simulink model "Guidance_HIL_XPlane"  (R2026b)
settings: Solver=ode4  StopTime=80  FixedStep=0.005  MaxStep=0.05  MinStep=1e-8  AbsTol=1e-4
StartFcn:
  | ins_initial_state_xplane;
undefined symbols (not defined in the file or in its folder): sensors
(part 1 of 2)
settings Model: Creator=anade  LastModifiedBy=julio
settings DataIOCC: SaveState=on

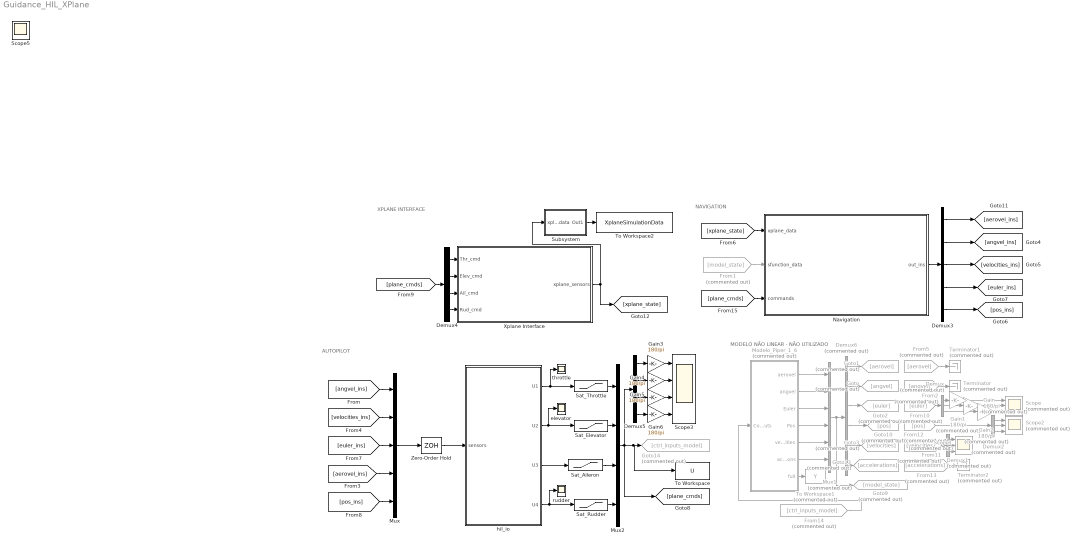
== system Guidance_HIL_XPlane ==
  note: MODELO NÃO LINEAR - NÃO UTILIZADO
  note: NAVIGATION
  note: AUTOPILOT
  note: XPLANE INTERFACE
  Demux : Demux  Commented=on  Outputs=3
  Demux1 : Demux  Commented=on  Outputs=3
  Demux2 : Demux  Commented=on  Outputs=3
  Demux3 : Demux  Outputs=5
  Demux4 : Demux
  Demux5 : Demux
  Demux6 : Demux  Commented=on  Outputs=6
  From1 : From  Commented=on  GotoTag=model_state
  From10 : From  Commented=on  GotoTag=euler
  From11 : From  Commented=on  GotoTag=velocities
  From12 : From  Commented=on  GotoTag=pos
  From13 : From  Commented=on  GotoTag=accelerations
  From14 : From  Commented=on  GotoTag=ctrl_inputs_model
  From2 : From  Commented=on  GotoTag=angvel
  From5 : From  Commented=on  GotoTag=aerovel
  Gain : Gain  Commented=on  Gain=180/pi
  Gain1 : Gain  Commented=on  Gain=180/pi
  Gain2 : Gain  Commented=on  Gain=180/pi
  Gain{3..6} (4 alike) : Gain  Gain=180/pi
  Goto : Goto  Commented=on  GotoTag=angvel
  Goto1 : Goto  Commented=on  GotoTag=aerovel
  Goto10 : Goto  Commented=on  GotoTag=pos
  Goto13 : Goto  Commented=on  GotoTag=accelerations
  Goto14 : Goto  Commented=on  GotoTag=ctrl_inputs_model
  Goto2 : Goto  Commented=on  GotoTag=euler
  Goto3 : Goto  Commented=on  GotoTag=velocities
  Goto9 : Goto  Commented=on  GotoTag=model_state
  Modelo_Piper_1_6 : Subsystem  Commented=on
  Mux : Mux  Inputs=5
  Mux1 : Mux  Commented=on  Inputs=6
  Mux2 : Mux
  Navigation : Subsystem
  Sat_Aileron : Saturate  UpperLimit=0.4363  LowerLimit=-0.4363
  Sat_Elevator : Saturate  UpperLimit=0.4363  LowerLimit=-0.4363
  Sat_Rudder : Saturate  UpperLimit=0.4363  LowerLimit=-0.4363
  Sat_Throttle : Saturate  UpperLimit=1  LowerLimit=0
  Scope : Scope  Commented=on  NumInputPorts=3
      settings: ActiveDisplayYMinimum=-6.98611  ActiveDisplayYMaximum=5.63762
  Scope1 : Scope  Commented=on  NumInputPorts=3
      settings: ActiveDisplayYMinimum=14.85385  ActiveDisplayYMaximum=15.01624
  Scope2 : Scope  Commented=on  NumInputPorts=3
      settings: ActiveDisplayYMinimum=-260.5736  ActiveDisplayYMaximum=2345.16236  DataLoggingVariableName=ScopeData4
  Scope3 : Scope  NumInputPorts=4
      settings: ActiveDisplayYMinimum=27.28743  ActiveDisplayYMaximum=28.20495
  Subsystem : Subsystem
  Terminator : Terminator  Commented=on
  Terminator1 : Terminator  Commented=on
  Terminator2 : Terminator  Commented=on
  To Workspace : ToWorkspace  VariableName=U  SaveFormat=Structure With Time  SampleTime=-1
  To Workspace1 : ToWorkspace  Commented=on  VariableName=Y  SaveFormat=Structure With Time  SampleTime=-1
  To Workspace2 : ToWorkspace  VariableName=XplaneSimulationData  SaveFormat=Structure With Time  SampleTime=-1
  Xplane Interface : Subsystem
  Zero-Order Hold : ZeroOrderHold  SampleTime=0.01
  elevator : Scope
      settings: ActiveDisplayYMinimum=-0.5444964451073081  ActiveDisplayYMaximum=0.59983808374051317  DataLoggingVariableName=ScopeData11
  hil_io : MATLAB Function  TreatAsAtomicUnit=on
  rudder : Scope
      settings: ActiveDisplayYMinimum=-0.082744402354985674  ActiveDisplayYMaximum=0.075589414066673855  DataLoggingVariableName=ScopeData9
  throttle : Scope
      settings: ActiveDisplayYMinimum=-0.079216538751602131  ActiveDisplayYMaximum=0.72681884876441949  DataLoggingVariableName=ScopeData10
  Scope5 : Scope
      settings: ActiveDisplayYMinimum=-10.063291139240507  ActiveDisplayYMaximum=10.936708860759492  DataLoggingVariableName=ScopeData6
  wires:
  Mux2/1 -> To Workspace/1, Goto14/1, [plane_cmds], Demux5/1
  Modelo_Piper_1_6/7(full) -> To Workspace1/1
  Demux/1 -> Gain1/1
  Demux/2 -> Gain/1
  Demux/3 -> Gain2/1
  Gain/1 -> Scope/2
  Demux1/1 -> Scope1/1
  Demux1/2 -> Scope1/2
  Demux1/3 -> Scope1/3
  Demux2/3 -> Scope2/3
  Demux2/2 -> Scope2/2
  Demux2/1 -> Scope2/1
  [aerovel_ins] -> Mux/4
  hil_io/1(U1) -> Sat_Throttle/1, throttle/1
  hil_io/2(U2) -> Sat_Elevator/1, elevator/1
  hil_io/3(U3) -> Sat_Aileron/1
  Gain1/1 -> Scope/1
  Gain2/1 -> Scope/3
  Gain3/1 -> Scope3/1
  Gain4/1 -> Scope3/2
  Gain5/1 -> Scope3/3
  Gain6/1 -> Scope3/4
  Sat_Throttle/1 -> Mux2/1
  Sat_Elevator/1 -> Mux2/2
  Sat_Aileron/1 -> Mux2/3
  Sat_Rudder/1 -> Mux2/4
  Demux3/2 -> [angvel_ins]
  Demux3/3 -> [velocities_ins]
  Demux3/4 -> [euler_ins]
  Demux3/5 -> [pos_ins]
  Navigation/1(out_ins) -> Demux3/1
  [angvel_ins] -> Mux/1
  [velocities_ins] -> Mux/2
  [euler_ins] -> Mux/3
  [pos_ins] -> Mux/5
  [plane_cmds] -> Demux4/1
  Demux4/1 -> Xplane Interface/1(Thr_cmd)
  Demux4/2 -> Xplane Interface/2(Elev_cmd)
  Demux4/3 -> Xplane Interface/3(Ail_cmd)
  Demux4/4 -> Xplane Interface/4(Rud_cmd)
  Demux5/1 -> Gain3/1
  Demux5/2 -> Gain4/1
  Demux5/3 -> Gain5/1
  Demux5/4 -> Gain6/1
  Modelo_Piper_1_6/1(aerovel) -> Mux1/1
  Modelo_Piper_1_6/2(angvel) -> Mux1/2
  Modelo_Piper_1_6/3(Euler) -> Mux1/3
  Modelo_Piper_1_6/4(Pos) -> Mux1/4
  Modelo_Piper_1_6/5(velocities) -> Mux1/5
  Demux6/1 -> Goto1/1
  Demux6/2 -> Goto/1
  Demux6/3 -> Goto2/1
  Demux6/4 -> Goto10/1
  Demux6/5 -> Goto3/1
  From2/1 -> Terminator/1
  Demux3/1 -> [aerovel_ins]
  From5/1 -> Terminator1/1
  From12/1 -> Demux2/1
  From10/1 -> Demux/1
  From11/1 -> Demux1/1
  Xplane Interface/1(xplane_sensors) -> Subsystem/1(xplane_data), [xplane_state]
  [xplane_state] -> Navigation/1(xplane_data)
  Modelo_Piper_1_6/6(accelerations) -> Mux1/6
  Mux1/1 -> Goto9/1, Demux6/1
  Demux6/6 -> Goto13/1
  From13/1 -> Terminator2/1
  hil_io/4(U4) -> Sat_Rudder/1, rudder/1
  Subsystem/1(Out1) -> To Workspace2/1
  From14/1 -> Modelo_Piper_1_6/1(Control Inputs)
  From1/1 -> Navigation/2(sfunction_data)
  [plane_cmds] -> Navigation/3(commands)
  Zero-Order Hold/1 -> hil_io/1(sensors)
  Mux/1 -> Zero-Order Hold/1

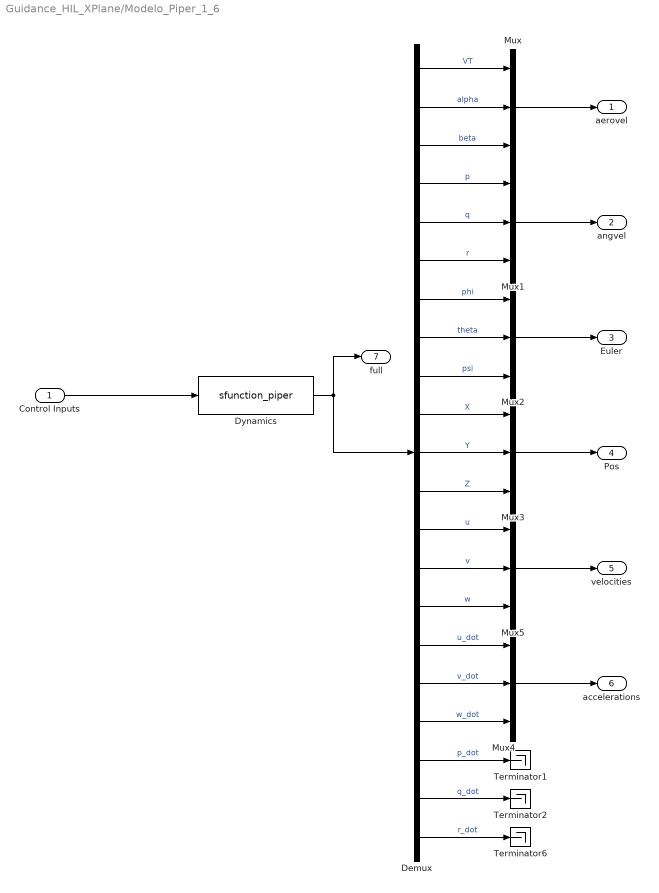
== system Guidance_HIL_XPlane/Modelo_Piper_1_6 ==
  Control Inputs : Inport
  Demux : Demux  Outputs=21
  Dynamics : S-Function  FunctionName=sfunction_piper  Parameters=par_gen,par_aero,par_prop, Xe  SFunctionDeploymentMode=off  EnableBusSupport=off
  Mux{,1..5} (6 alike) : Mux  Inputs=3
  Terminator1 : Terminator
  Terminator2 : Terminator
  Terminator6 : Terminator
  aerovel : Outport
  angvel : Outport  Port=2
  Euler : Outport  Port=3
  Pos : Outport  Port=4
  velocities : Outport  Port=5
  accelerations : Outport  Port=6
  full : Outport  Port=7
  wires:
  Control Inputs/1 -> Dynamics/1
  Dynamics/1 -> full/1, Demux/1
  Demux/1 -> Mux/1  "VT"
  Demux/2 -> Mux/2  "alpha"
  Demux/3 -> Mux/3  "beta"
  Mux/1 -> aerovel/1
  Demux/6 -> Mux1/3  "r"
  Demux/4 -> Mux1/1  "p"
  Mux1/1 -> angvel/1
  Demux/5 -> Mux1/2  "q"
  Mux2/1 -> Euler/1
  Demux/9 -> Mux2/3  "psi"
  Demux/7 -> Mux2/1  "phi"
  Demux/8 -> Mux2/2  "theta"
  Demux/11 -> Mux3/2  "Y"
  Demux/10 -> Mux3/1  "X"
  Demux/12 -> Mux3/3  "Z"
  Mux3/1 -> Pos/1
  Demux/14 -> Mux5/2  "v"
  Demux/15 -> Mux5/3  "w"
  Demux/17 -> Mux4/2  "v_dot"
  Demux/18 -> Mux4/3  "w_dot"
  Demux/16 -> Mux4/1  "u_dot"
  Demux/19 -> Terminator1/1  "p_dot"
  Demux/20 -> Terminator2/1  "q_dot"
  Demux/21 -> Terminator6/1  "r_dot"
  Demux/13 -> Mux5/1  "u"
  Mux5/1 -> velocities/1
  Mux4/1 -> accelerations/1

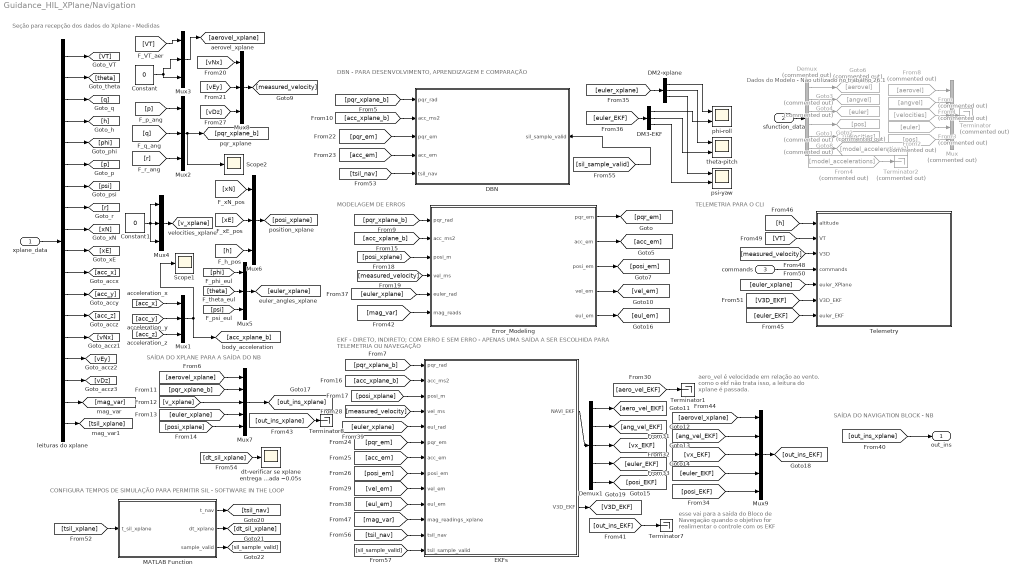
== system Guidance_HIL_XPlane/Navigation ==
  note: CONFIGURA TEMPOS DE SIMULAÇÃO PARA PERMITIR
      | SIL - SOFTWARE IN THE LOOP
  note: DBN - PARA DESENVOLVIMENTO, APRENDIZAGEM E COMPARAÇÃO
  note: MODELAGEM DE ERROS
  note: EKF - DIRETO, INDIRETO; COM ERRO E SEM ERRO - APENAS UMA SAÍDA A SER ESCOLHIDA PARA TELEMETRIA OU NAVEGAÇÃO
  note: TELEMETRIA PARA O CLI
  note: aero_vel é velocidade em relação ao vento.
      | como o ekf não trata isso, a leitura do xplane é passada.
  note: SAÍDA DO NAVIGATION BLOCK - NB
  note: SAÍDA DO XPLANE PARA A SAÍDA DO NB
  note: Seção para recepção dos dados do Xplane - Medidas
  note: Dados do Modelo - Não utilizado no trabalho 26.1
  note: esse vai para a saída do
      | Bloco de Navegação quando o objetivo
      | for realimentar o controle com os EKF
  xplane_data : Inport
  sfunction_data : Inport  Port=2
  commands : Inport  Port=3
  Constant : Constant  Value=0
  Constant1 : Constant  Value=0
  DBN : Subsystem
      settings: PortSchema="{\"entries\":[{\"content\":{\"sides\":[{\"content\":{\"connectorIds\":[\"In1\",\"In2\",\"In3\",\"In4\",\"In5\"]},\"type\":\"ConnectorPlacement.EquallySpacedRectSide\",\"uuid\":\"e1d6fc02-7142-43fa-9a22-3751041ad3ea\"},{\"content\":{\"connectorIds\":[\"In6\"],\"side\":\"RIGHT\"},\"type\":\"ConnectorPlacement.EquallySpacedRectSide\",\"uuid\":\"c1701565-012f-4813-aa31-4d1b787e29e9\"},{\"content\":{\"side\":\"TOP\"},\"type\":\"ConnectorPlacement.EquallySpacedRectSide\",\"uuid\":\"7000accd-9525-4039-8d3a-2953233d8ced\"},{\"content\":{\"side\":\"BOTTOM\"},\"type\":\"ConnectorPlacement.EquallySpacedRectSide\",\"uuid\":\"71202a87-1554-4160-a726-314bf509973f\"}]},\"type\":\"ConnectorPlacement.EquallySpacedConnector\",\"uuid\":\"ce59d3ba-4702-4e8e-9706-d7679f847eab\"}],\"packageUris\":[\"http://schema.mathworks.com/mf0/Connector/R2020b\"],\"version\":\"1.0\"}"
  DM2-xplane : Demux  Outputs=3
  DM3-EKF : Demux  Outputs=3
  Demux : Demux  Commented=on  Outputs=6
  Demux1 : Demux  Outputs=5
  EKFs : Subsystem
  Error_Modeling : Subsystem
  From : From  Commented=on  GotoTag=angvel
  From1 : From  Commented=on  GotoTag=velocities
  From2 : From  Commented=on  GotoTag=euler
  From3 : From  Commented=on  GotoTag=pos
  From4 : From  Commented=on  GotoTag=model_accelerations
  From8 : From  Commented=on  GotoTag=aerovel
  Goto1 : Goto  Commented=on  GotoTag=velocities
  Goto2 : Goto  Commented=on  GotoTag=pos
  Goto3 : Goto  Commented=on  GotoTag=angvel
  Goto4 : Goto  Commented=on  GotoTag=euler
  Goto6 : Goto  Commented=on  GotoTag=aerovel
  Goto8 : Goto  Commented=on  GotoTag=model_accelerations
  MATLAB Function : MATLAB Function  TreatAsAtomicUnit=on
  Mux : Mux  Commented=on  Inputs=5
  Mux{1..6,8} (7 alike) : Mux  Inputs=3
  Mux7 : Mux  Inputs=5
  Mux9 : Mux  Inputs=5
  Scope1 : Scope
      settings: ActiveDisplayYMinimum=-16.174539597742694  ActiveDisplayYMaximum=12.212616009640644  DataLoggingVariableName=ScopeData7
  Scope2 : Scope
      settings: DataLoggingVariableName=ScopeData8
  Telemetry : Subsystem
  Terminator : Terminator  Commented=on
  Terminator1 : Terminator
  Terminator2 : Terminator  Commented=on
  Terminator7 : Terminator
  Terminator8 : Terminator
  dt-verificar se xplane entrega a cada ~0.05s : Scope
      settings: ActiveDisplayYMinimum=-39.174751163951377  ActiveDisplayYMaximum=35.494375282880192  DataLoggingVariableName=ScopeData18
  leituras do xplane : Demux  Outputs=18
  phi-roll : Scope  NumInputPorts=2
      settings: ActiveDisplayYMinimum=-36.313013678398512  ActiveDisplayYMaximum=32.517817448050167  DataLoggingVariableName=ScopeData13
  psi-yaw : Scope  NumInputPorts=2
      settings: ActiveDisplayYMinimum=-3.9264088034500482  ActiveDisplayYMaximum=3.9263427428668405  DataLoggingVariableName=ScopeData17
  theta-pitch : Scope  NumInputPorts=2
      settings: ActiveDisplayYMinimum=-1.9059189366815974  ActiveDisplayYMaximum=3.346694670659121  DataLoggingVariableName=ScopeData16
  out_ins : Outport
  wires:
  xplane_data/1 -> leituras do xplane/1
  leituras do xplane/1 -> [VT]
  leituras do xplane/6 -> [p]
  leituras do xplane/9 -> [xN]
  leituras do xplane/3 -> [q]
  leituras do xplane/8 -> [r]
  leituras do xplane/5 -> [phi]
  leituras do xplane/10 -> [xE]
  leituras do xplane/2 -> [theta]
  leituras do xplane/7 -> [psi]
  leituras do xplane/4 -> [h]
  leituras do xplane/11 -> [acc_x]
  leituras do xplane/12 -> [acc_y]
  leituras do xplane/13 -> [acc_z]
  [VT] -> Mux3/1
  [p] -> Mux2/1
  [r] -> Mux2/3
  [acc_x] -> Mux1/1
  [acc_y] -> Mux1/2
  [acc_z] -> Mux1/3
  Mux1/1 -> Scope1/1, [acc_xplane_b]
  Mux2/1 -> [pqr_xplane_b], Scope2/1
  [q] -> Mux2/2
  Constant/1 -> Mux3/2, Mux3/3
  Mux3/1 -> [aerovel_xplane]
  Constant1/1 -> Mux4/3, Mux4/1, Mux4/2
  Mux4/1 -> [v_xplane]
  Mux5/1 -> [euler_xplane]
  [phi] -> Mux5/1
  [theta] -> Mux5/2
  [psi] -> Mux5/3
  [xN] -> Mux6/1
  [xE] -> Mux6/2
  [h] -> Mux6/3
  Mux6/1 -> [posi_xplane]
  [aerovel_xplane] -> Mux7/1
  [pqr_xplane_b] -> Mux7/2
  [v_xplane] -> Mux7/3
  [euler_xplane] -> Mux7/4
  [posi_xplane] -> Mux7/5
  [pqr_xplane_b] -> DBN/1(pqr_rad)
  [acc_xplane_b] -> DBN/2(acc_ms2)
  Error_Modeling/1(pqr_em) -> [pqr_em]
  Error_Modeling/2(acc_em) -> [acc_em]
  Error_Modeling/3(posi_em) -> [posi_em]
  [pqr_xplane_b] -> EKFs/1(pqr_rad)
  [acc_xplane_b] -> EKFs/2(acc_ms2)
  [posi_xplane] -> EKFs/3(posi_m)
  [pqr_xplane_b] -> Error_Modeling/1(pqr_rad)
  [acc_xplane_b] -> Error_Modeling/2(acc_ms2)
  [posi_xplane] -> Error_Modeling/3(posi_m)
  [pqr_em] -> DBN/3(pqr_em)
  [acc_em] -> DBN/4(acc_em)
  [measured_velocity] -> EKFs/4(vel_ms)
  [pqr_em] -> EKFs/6(pqr_em)
  [acc_em] -> EKFs/7(acc_em)
  [posi_em] -> EKFs/8(posi_em)
  leituras do xplane/14 -> [vNx]
  leituras do xplane/15 -> [vEy]
  leituras do xplane/16 -> [vDz]
  [vNx] -> Mux8/1
  [vEy] -> Mux8/2
  [vDz] -> Mux8/3
  Mux8/1 -> [measured_velocity]
  [measured_velocity] -> Error_Modeling/4(vel_ms)
  Error_Modeling/4(vel_em) -> [vel_em]
  [vel_em] -> EKFs/9(vel_em)
  Demux1/1 -> [aero_vel_EKF]
  Demux1/2 -> [ang_vel_EKF]
  Demux1/3 -> [vx_EKF]
  Demux1/4 -> [euler_EKF]
  Demux1/5 -> [posi_EKF]
  [aero_vel_EKF] -> Terminator1/1
  [ang_vel_EKF] -> Mux9/2
  [vx_EKF] -> Mux9/3
  [euler_EKF] -> Mux9/4
  [posi_EKF] -> Mux9/5
  [euler_xplane] -> DM2-xplane/1
  DM2-xplane/1 -> phi-roll/1
  DM2-xplane/2 -> theta-pitch/1
  DM2-xplane/3 -> psi-yaw/1
  [euler_EKF] -> DM3-EKF/1
  DM3-EKF/1 -> phi-roll/2
  DM3-EKF/2 -> theta-pitch/2
  DM3-EKF/3 -> psi-yaw/2
  Demux/5 -> Goto1/1
  Mux/1 -> Terminator/1
  From8/1 -> Mux/1
  Demux/6 -> Goto8/1
  Demux/1 -> Goto6/1
  Demux/2 -> Goto3/1
  From/1 -> Mux/2
  From3/1 -> Mux/5
  From4/1 -> Terminator2/1
  Demux/3 -> Goto4/1
  From2/1 -> Mux/4
  Demux/4 -> Goto2/1
  From1/1 -> Mux/3
  sfunction_data/1 -> Demux/1
  [euler_xplane] -> Error_Modeling/5(euler_rad)
  Error_Modeling/5(eul_em) -> [eul_em]
  [eul_em] -> EKFs/10(eul_em)
  [euler_xplane] -> EKFs/5(eul_rad)
  Mux7/1 -> [out_ins_xplane]
  [out_ins_xplane] -> out_ins/1
  EKFs/1(NAVI_EKF) -> Demux1/1
  [out_ins_EKF] -> Terminator7/1
  [out_ins_xplane] -> Terminator8/1
  leituras do xplane/17 -> [mag_var]
  [mag_var] -> EKFs/11(mag_readings_xplane)
  [mag_var] -> Error_Modeling/6(mag_reads)
  Mux9/1 -> [out_ins_EKF]
  [aerovel_xplane] -> Mux9/1
  commands/1 -> Telemetry/4(commands)
  [h] -> Telemetry/1(altitude)
  [measured_velocity] -> Telemetry/3(V3D)
  [VT] -> Telemetry/2(VT)
  [euler_xplane] -> Telemetry/5(euler_XPlane)
  [euler_EKF] -> Telemetry/7(euler_EKF)
  EKFs/2(V3D_EKF) -> [V3D_EKF]
  [V3D_EKF] -> Telemetry/6(V3D_EKF)
  leituras do xplane/18 -> [tsil_xplane]
  [tsil_xplane] -> MATLAB Function/1(t_sil_xplane)
  MATLAB Function/2(dt_xplane) -> [dt_sil_xplane]
  MATLAB Function/1(t_nav) -> [tsil_nav]
  MATLAB Function/3(sample_valid) -> [sil_sample_valid]
  [tsil_nav] -> DBN/5(tsil_nav)
  [sil_sample_valid] -> DBN/6(sil_sample_valid)
  [dt_sil_xplane] -> dt-verificar se xplane entrega a cada ~0.05s/1
  [tsil_nav] -> EKFs/12(tsil_nav)
  [sil_sample_valid] -> EKFs/13(tsil_sample_valid)

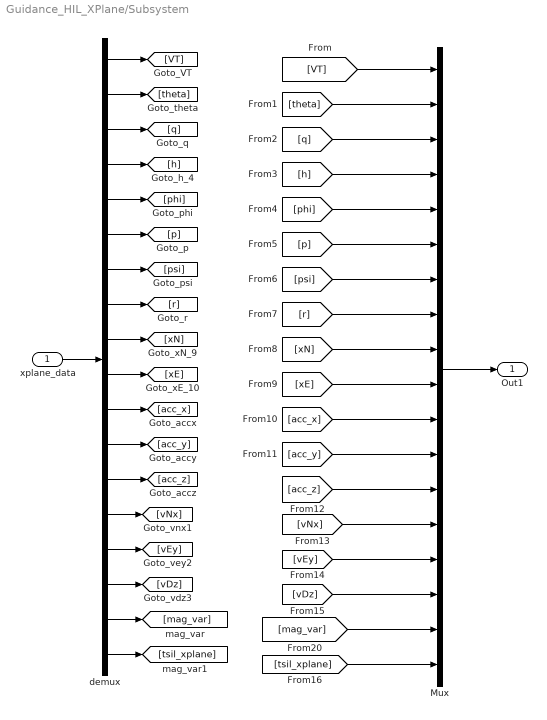
== system Guidance_HIL_XPlane/Subsystem ==
  xplane_data : Inport
  Mux : Mux  Inputs=18
  demux : Demux  Outputs=18
  Out1 : Outport
  wires:
  demux/3 -> [q]
  demux/8 -> [r]
  demux/4 -> [h]
  demux/2 -> [theta]
  demux/6 -> [p]
  demux/1 -> [VT]
  xplane_data/1 -> demux/1
  demux/9 -> [xN]
  demux/12 -> [acc_y]
  demux/11 -> [acc_x]
  demux/13 -> [acc_z]
  demux/10 -> [xE]
  demux/7 -> [psi]
  demux/5 -> [phi]
  [VT] -> Mux/1
  [theta] -> Mux/2
  [q] -> Mux/3
  [h] -> Mux/4
  [phi] -> Mux/5
  [p] -> Mux/6
  [psi] -> Mux/7
  [r] -> Mux/8
  [xN] -> Mux/9
  [xE] -> Mux/10
  [acc_x] -> Mux/11
  [acc_y] -> Mux/12
  [acc_z] -> Mux/13
  Mux/1 -> Out1/1
  demux/14 -> [vNx]
  demux/15 -> [vEy]
  demux/16 -> [vDz]
  [vNx] -> Mux/14
  [vEy] -> Mux/15
  [vDz] -> Mux/16
  [mag_var] -> Mux/17
  demux/17 -> [mag_var]
  demux/18 -> [tsil_xplane]
  [tsil_xplane] -> Mux/18

== system Guidance_HIL_XPlane/Xplane Interface ==
  Thr_cmd : Inport
  Elev_cmd : Inport  Port=2
  Ail_cmd : Inport  Port=3
  Rud_cmd : Inport  Port=4
  Clock : Clock
  Cmd Mux : Mux
  Terminator : Terminator
  X-Plane Actuators : MATLAB Function  TreatAsAtomicUnit=on
  X-Plane Sensors : MATLAB Function  TreatAsAtomicUnit=on
  Zero-Order Hold : ZeroOrderHold  SampleTime=0.01
  xplane_sensors : Outport
  wires:
  Cmd Mux/1 -> Zero-Order Hold/1
  Elev_cmd/1 -> Cmd Mux/1
  Ail_cmd/1 -> Cmd Mux/2
  Rud_cmd/1 -> Cmd Mux/3
  Thr_cmd/1 -> Cmd Mux/4
  Clock/1 -> X-Plane Sensors/1(t), X-Plane Actuators/2(t)
  X-Plane Actuators/1(status) -> Terminator/1
  Zero-Order Hold/1 -> X-Plane Actuators/1(u)
  X-Plane Sensors/1(xplane_sensors) -> xplane_sensors/1

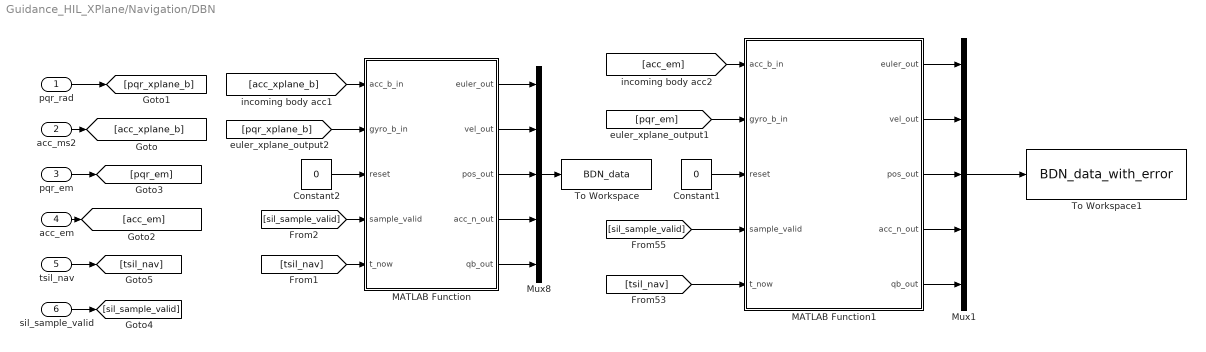
== system Guidance_HIL_XPlane/Navigation/DBN ==
  pqr_rad : Inport
  acc_ms2 : Inport  Port=2
  pqr_em : Inport  Port=3
  acc_em : Inport  Port=4
  tsil_nav : Inport  Port=5
  sil_sample_valid : Inport  Port=6
  Constant1 : Constant  Value=0
  Constant2 : Constant  Value=0
  MATLAB Function : MATLAB Function  TreatAsAtomicUnit=on
  MATLAB Function1 : MATLAB Function  TreatAsAtomicUnit=on
  Mux1 : Mux  Inputs=5
  Mux8 : Mux  Inputs=5
  To Workspace : ToWorkspace  VariableName=BDN_data  SaveFormat=Structure With Time  SampleTime=-1
  To Workspace1 : ToWorkspace  VariableName=BDN_data_with_error  SaveFormat=Structure With Time  SampleTime=-1
  wires:
  Constant2/1 -> MATLAB Function/3(reset)
  MATLAB Function/2(vel_out) -> Mux8/2
  MATLAB Function/1(euler_out) -> Mux8/1
  MATLAB Function/4(acc_n_out) -> Mux8/4
  MATLAB Function/5(qb_out) -> Mux8/5
  MATLAB Function/3(pos_out) -> Mux8/3
  Mux8/1 -> To Workspace/1
  [acc_xplane_b] -> MATLAB Function/1(acc_b_in)
  [pqr_xplane_b] -> MATLAB Function/2(gyro_b_in)
  acc_ms2/1 -> [acc_xplane_b]
  pqr_rad/1 -> [pqr_xplane_b]
  [pqr_em] -> MATLAB Function1/2(gyro_b_in)
  [acc_em] -> MATLAB Function1/1(acc_b_in)
  [tsil_nav] -> MATLAB Function1/5(t_now)
  Mux1/1 -> To Workspace1/1
  MATLAB Function1/3(pos_out) -> Mux1/3
  MATLAB Function1/5(qb_out) -> Mux1/5
  MATLAB Function1/2(vel_out) -> Mux1/2
  MATLAB Function1/4(acc_n_out) -> Mux1/4
  [sil_sample_valid] -> MATLAB Function1/4(sample_valid)
  MATLAB Function1/1(euler_out) -> Mux1/1
  Constant1/1 -> MATLAB Function1/3(reset)
  acc_em/1 -> [acc_em]
  pqr_em/1 -> [pqr_em]
  sil_sample_valid/1 -> [sil_sample_valid]
  tsil_nav/1 -> [tsil_nav]
  [tsil_nav] -> MATLAB Function/5(t_now)
  [sil_sample_valid] -> MATLAB Function/4(sample_valid)

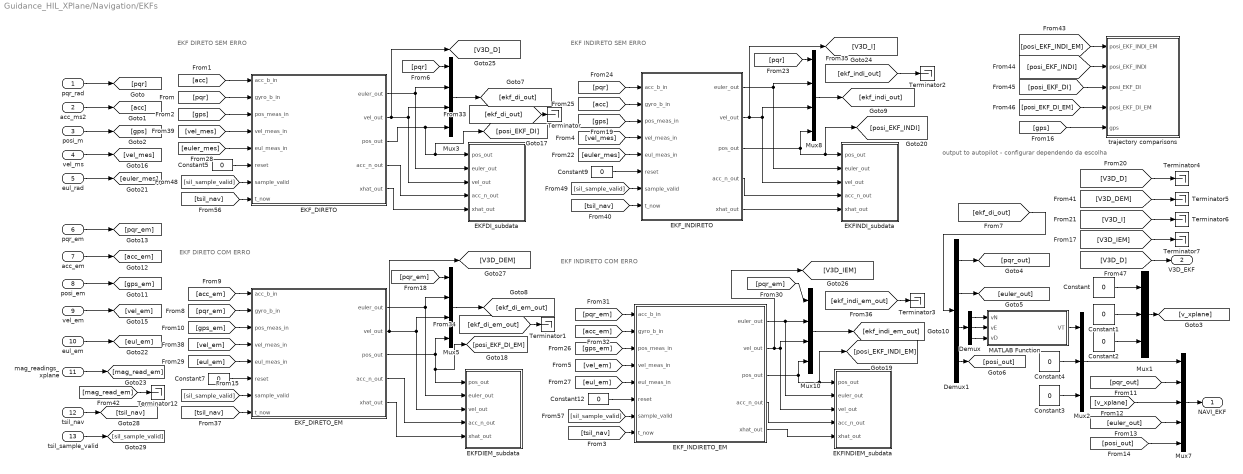
== system Guidance_HIL_XPlane/Navigation/EKFs ==
  note: EKF INDIRETO COM ERRO
  note: EKF INDIRETO SEM ERRO
  note: EKF DIRETO COM ERRO
  note: EKF DIRETO SEM ERRO
  note: output to autopilot - configurar dependendo da escolha
  pqr_rad : Inport
  acc_ms2 : Inport  Port=2
  posi_m : Inport  Port=3
  vel_ms : Inport  Port=4
  eul_rad : Inport  Port=5
  pqr_em : Inport  Port=6
  acc_em : Inport  Port=7
  posi_em : Inport  Port=8
  vel_em : Inport  Port=9
  eul_em : Inport  Port=10
  mag_readings_xplane : Inport  Port=11
  tsil_nav : Inport  Port=12
  tsil_sample_valid : Inport  Port=13
  Constant{,1..5,7,9,12} (9 alike) : Constant  Value=0
  Demux : Demux  Outputs=3
  Demux1 : Demux
  EKFDIEM_subdata : Subsystem
  EKFDI_subdata : Subsystem
  EKFINDIEM_subdata : Subsystem
  EKFINDI_subdata : Subsystem
  EKF_DIRETO : MATLAB Function  TreatAsAtomicUnit=on
  EKF_DIRETO_EM : MATLAB Function  TreatAsAtomicUnit=on
  EKF_INDIRETO : MATLAB Function  TreatAsAtomicUnit=on
  EKF_INDIRETO_EM : MATLAB Function  TreatAsAtomicUnit=on
  MATLAB Function : MATLAB Function  TreatAsAtomicUnit=on
  Mux1 : Mux  Inputs=3
  Mux{3,5,8,10} (4 alike) : Mux
  Mux2 : Mux  Inputs=3
  Mux7 : Mux  Inputs=5
  Terminator{,1..7,12} (9 alike) : Terminator
  trajectory comparisons : Subsystem
  NAVI_EKF : Outport
  V3D_EKF : Outport  Port=2
  wires:
  EKF_DIRETO/3(pos_out) -> Mux3/4, EKFDI_subdata/1(pos_out), [posi_EKF_DI]
  posi_m/1 -> [gps]
  acc_ms2/1 -> [acc]
  pqr_rad/1 -> [pqr]
  [gps] -> EKF_DIRETO/3(pos_meas_in)
  Mux7/1 -> NAVI_EKF/1
  [posi_out] -> Mux7/5
  [v_xplane] -> Mux7/3
  [pqr_out] -> Mux7/2
  [euler_out] -> Mux7/4
  Mux1/1 -> [v_xplane]
  Constant/1 -> Mux1/1
  Constant2/1 -> Mux1/3
  Constant1/1 -> Mux1/2
  Demux/1 -> MATLAB Function/1(vN)
  Demux/2 -> MATLAB Function/2(vE)
  Demux/3 -> MATLAB Function/3(vD)
  MATLAB Function/1(VT) -> Mux2/1
  Constant4/1 -> Mux2/2
  Constant3/1 -> Mux2/3
  Mux2/1 -> Mux7/1
  Demux1/4 -> [posi_out]
  Mux3/1 -> [ekf_di_out]
  [ekf_di_out] -> Demux1/1
  [gps_em] -> EKF_DIRETO_EM/3(pos_meas_in)
  EKF_DIRETO_EM/3(pos_out) -> [posi_EKF_DI_EM], EKFDIEM_subdata/1(pos_out), Mux5/4
  EKF_DIRETO_EM/1(euler_out) -> Mux5/2, EKFDIEM_subdata/2(euler_out)
  Mux5/1 -> [ekf_di_em_out]
  Mux8/1 -> [ekf_indi_out]
  [pqr] -> EKF_INDIRETO/1(acc_b_in)
  EKF_INDIRETO/3(pos_out) -> Mux8/4, [posi_EKF_INDI], EKFINDI_subdata/1(pos_out)
  [gps] -> EKF_INDIRETO/3(pos_meas_in)
  [acc] -> EKF_INDIRETO/2(gyro_b_in)
  [acc_em] -> EKF_INDIRETO_EM/2(gyro_b_in)
  [gps_em] -> EKF_INDIRETO_EM/3(pos_meas_in)
  [pqr_em] -> EKF_INDIRETO_EM/1(acc_b_in)
  Mux10/1 -> [ekf_indi_em_out]
  [ekf_di_out] -> Terminator/1
  [ekf_di_em_out] -> Terminator1/1
  [ekf_indi_out] -> Terminator2/1
  [ekf_indi_em_out] -> Terminator3/1
  [tsil_nav] -> EKF_DIRETO/8(t_now)
  Constant5/1 -> EKF_DIRETO/6(reset)
  pqr_em/1 -> [pqr_em]
  acc_em/1 -> [acc_em]
  posi_em/1 -> [gps_em]
  vel_em/1 -> [vel_em]
  vel_ms/1 -> [vel_mes]
  [vel_mes] -> EKF_DIRETO/4(vel_meas_in)
  [acc_em] -> EKF_DIRETO_EM/1(acc_b_in)
  [pqr_em] -> EKF_DIRETO_EM/2(gyro_b_in)
  [vel_em] -> EKF_DIRETO_EM/4(vel_meas_in)
  [pqr] -> EKF_DIRETO/2(gyro_b_in)
  [acc] -> EKF_DIRETO/1(acc_b_in)
  Constant7/1 -> EKF_DIRETO_EM/6(reset)
  EKF_DIRETO/4(acc_n_out) -> EKFDI_subdata/4(acc_n_out)
  EKF_DIRETO/5(xhat_out) -> EKFDI_subdata/5(xhat_out)
  [pqr] -> Mux3/1
  EKF_DIRETO/1(euler_out) -> Mux3/2, EKFDI_subdata/2(euler_out)
  EKF_DIRETO/2(vel_out) -> [V3D_D], Mux3/3, EKFDI_subdata/3(vel_out)
  EKF_DIRETO_EM/5(xhat_out) -> EKFDIEM_subdata/5(xhat_out)
  Demux1/3 -> Demux/1
  Demux1/1 -> [pqr_out]
  Demux1/2 -> [euler_out]
  [pqr_em] -> Mux5/1
  EKF_DIRETO_EM/2(vel_out) -> Mux5/3, EKFDIEM_subdata/3(vel_out), [V3D_DEM]
  EKF_DIRETO_EM/4(acc_n_out) -> EKFDIEM_subdata/4(acc_n_out)
  [pqr] -> Mux8/1
  Constant9/1 -> EKF_INDIRETO/6(reset)
  [vel_mes] -> EKF_INDIRETO/4(vel_meas_in)
  EKF_INDIRETO/5(xhat_out) -> EKFINDI_subdata/5(xhat_out)
  EKF_INDIRETO/4(acc_n_out) -> EKFINDI_subdata/4(acc_n_out)
  EKF_INDIRETO/1(euler_out) -> Mux8/2, EKFINDI_subdata/2(euler_out)
  EKF_INDIRETO/2(vel_out) -> [V3D_I], Mux8/3, EKFINDI_subdata/3(vel_out)
  [pqr_em] -> Mux10/1
  EKF_INDIRETO_EM/1(euler_out) -> Mux10/2, EKFINDIEM_subdata/2(euler_out)
  EKF_INDIRETO_EM/2(vel_out) -> [V3D_IEM], Mux10/3, EKFINDIEM_subdata/3(vel_out)
  EKF_INDIRETO_EM/3(pos_out) -> Mux10/4, [posi_EKF_INDI_EM], EKFINDIEM_subdata/1(pos_out)
  [vel_em] -> EKF_INDIRETO_EM/4(vel_meas_in)
  Constant12/1 -> EKF_INDIRETO_EM/6(reset)
  EKF_INDIRETO_EM/4(acc_n_out) -> EKFINDIEM_subdata/4(acc_n_out)
  EKF_INDIRETO_EM/5(xhat_out) -> EKFINDIEM_subdata/5(xhat_out)
  eul_rad/1 -> [euler_mes]
  eul_em/1 -> [eul_em]
  [euler_mes] -> EKF_DIRETO/5(eul_meas_in)
  [eul_em] -> EKF_DIRETO_EM/5(eul_meas_in)
  [euler_mes] -> EKF_INDIRETO/5(eul_meas_in)
  [eul_em] -> EKF_INDIRETO_EM/5(eul_meas_in)
  mag_readings_xplane/1 -> [mag_read_em]
  [mag_read_em] -> Terminator12/1
  [posi_EKF_INDI_EM] -> trajectory comparisons/1(posi_EKF_INDI_EM)
  [posi_EKF_INDI] -> trajectory comparisons/2(posi_EKF_INDI)
  [posi_EKF_DI] -> trajectory comparisons/3(posi_EKF_DI)
  [posi_EKF_DI_EM] -> trajectory comparisons/4(posi_EKF_DI_EM)
  [gps] -> trajectory comparisons/5(gps)
  [V3D_D] -> Terminator4/1
  [V3D_DEM] -> Terminator5/1
  [V3D_I] -> Terminator6/1
  [V3D_IEM] -> Terminator7/1
  [V3D_D] -> V3D_EKF/1
  tsil_nav/1 -> [tsil_nav]
  tsil_sample_valid/1 -> [sil_sample_valid]
  [tsil_nav] -> EKF_DIRETO_EM/8(t_now)
  [tsil_nav] -> EKF_INDIRETO/8(t_now)
  [sil_sample_valid] -> EKF_INDIRETO_EM/7(sample_valid)
  [tsil_nav] -> EKF_INDIRETO_EM/8(t_now)
  [sil_sample_valid] -> EKF_DIRETO_EM/7(sample_valid)
  [sil_sample_valid] -> EKF_DIRETO/7(sample_valid)
  [sil_sample_valid] -> EKF_INDIRETO/7(sample_valid)

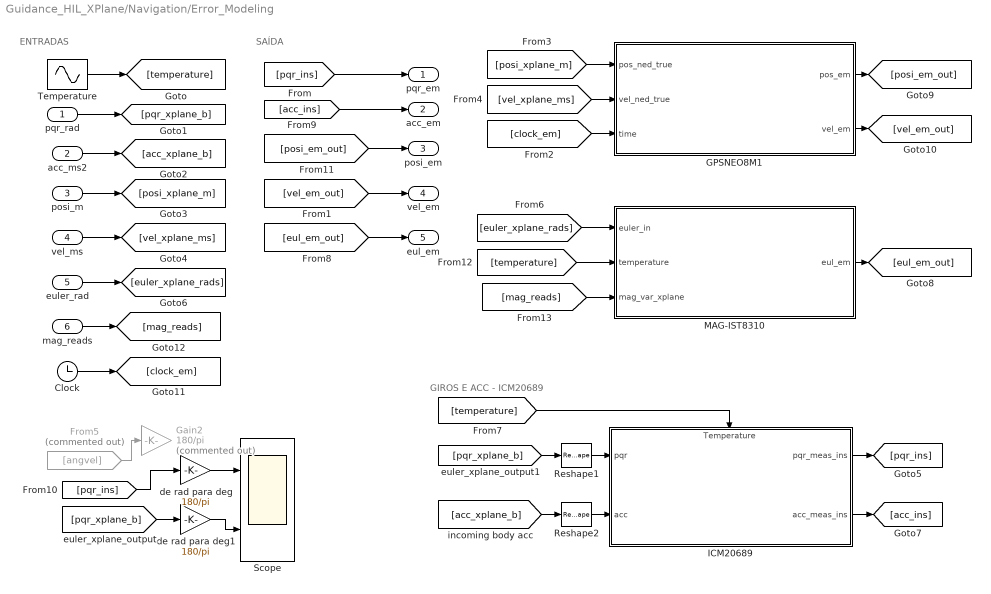
== system Guidance_HIL_XPlane/Navigation/Error_Modeling ==
  note: GIROS E ACC - ICM20689
  note: ENTRADAS
  note: SAÍDA
  pqr_rad : Inport
  acc_ms2 : Inport  Port=2
  posi_m : Inport  Port=3
  vel_ms : Inport  Port=4
  euler_rad : Inport  Port=5
  mag_reads : Inport  Port=6
  Clock : Clock
  From5 : From  Commented=on  GotoTag=angvel
  GPSNEO8M1 : Subsystem
  Gain2 : Gain  Commented=on  Gain=180/pi
  ICM20689 : Subsystem
      settings: PortSchema="{\"entries\":[{\"content\":{\"sides\":[{\"content\":{\"connectorIds\":[\"In1\",\"In2\"]},\"type\":\"ConnectorPlacement.EquallySpacedRectSide\",\"uuid\":\"9b78a035-9d4a-478e-9dc9-dc0bea5c931a\"},{\"content\":{\"connectorIds\":[\"Out1\",\"Out2\"],\"side\":\"RIGHT\"},\"type\":\"ConnectorPlacement.EquallySpacedRectSide\",\"uuid\":\"e21d77f8-fafe-45cf-b395-99fef016bd99\"},{\"content\":{\"connectorIds\":[\"In3\"],\"side\":\"TOP\"},\"type\":\"ConnectorPlacement.EquallySpacedRectSide\",\"uuid\":\"145a04c5-db60-4d84-a30a-895cdbce0dc0\"},{\"content\":{\"side\":\"BOTTOM\"},\"type\":\"ConnectorPlacement.EquallySpacedRectSide\",\"uuid\":\"826403f1-12d1-4d95-a630-f2fb059454f4\"}]},\"type\":\"ConnectorPlacement.EquallySpacedConnector\",\"uuid\":\"784d3b4a-97ce-487c-94bc-bef96ce83330\"}],\"packageUris\":[\"http://schema.mathworks.com/mf0/Connector/R2020b\"],\"version\":\"1.0\"}"
  MAG-IST8310 : Subsystem
  Reshape1 : Reshape  OutputDimensionality=Customize  OutputDimensions=[3 1]
  Reshape2 : Reshape  OutputDimensionality=Customize  OutputDimensions=[3 1]
  Scope : Scope  NumInputPorts=2
      settings: ActiveDisplayYMinimum=-72.109974321160792  ActiveDisplayYMaximum=81.22468249036686
  Temperature : Sin  Amplitude=10  Bias=25  Frequency=2*pi*0.01  SampleTime=0
  de rad para deg : Gain  Gain=180/pi
  de rad para deg1 : Gain  Gain=180/pi
  pqr_em : Outport
  acc_em : Outport  Port=2
  posi_em : Outport  Port=3
  vel_em : Outport  Port=4
  eul_em : Outport  Port=5
  wires:
  Reshape2/1 -> ICM20689/2(acc)
  de rad para deg/1 -> Scope/1
  ICM20689/1(pqr_meas_ins) -> [pqr_ins]
  [acc_ins] -> acc_em/1
  [pqr_ins] -> de rad para deg/1
  ICM20689/2(acc_meas_ins) -> [acc_ins]
  [acc_xplane_b] -> Reshape2/1
  From5/1 -> Gain2/1
  [temperature] -> ICM20689/3(Temperature)
  [pqr_xplane_b] -> Reshape1/1
  Reshape1/1 -> ICM20689/1(pqr)
  Temperature/1 -> [temperature]
  pqr_rad/1 -> [pqr_xplane_b]
  acc_ms2/1 -> [acc_xplane_b]
  [pqr_ins] -> pqr_em/1
  posi_m/1 -> [posi_xplane_m]
  [posi_em_out] -> posi_em/1
  [pqr_xplane_b] -> de rad para deg1/1
  de rad para deg1/1 -> Scope/2
  vel_ms/1 -> [vel_xplane_ms]
  [vel_em_out] -> vel_em/1
  [posi_xplane_m] -> GPSNEO8M1/1(pos_ned_true)
  [vel_xplane_ms] -> GPSNEO8M1/2(vel_ned_true)
  euler_rad/1 -> [euler_xplane_rads]
  [euler_xplane_rads] -> MAG-IST8310/1(euler_in)
  MAG-IST8310/1(eul_em) -> [eul_em_out]
  [eul_em_out] -> eul_em/1
  GPSNEO8M1/1(pos_em) -> [posi_em_out]
  GPSNEO8M1/2(vel_em) -> [vel_em_out]
  Clock/1 -> [clock_em]
  [clock_em] -> GPSNEO8M1/3(time)
  [temperature] -> MAG-IST8310/2(temperature)
  mag_reads/1 -> [mag_reads]
  [mag_reads] -> MAG-IST8310/3(mag_var_xplane)

== system Guidance_HIL_XPlane/Navigation/Telemetry ==
  altitude : Inport
  VT : Inport  Port=2
  V3D : Inport  Port=3
  commands : Inport  Port=4
  euler_XPlane : Inport  Port=5
  V3D_EKF : Inport  Port=6
  euler_EKF : Inport  Port=7
  Clock : Clock
  MATLAB Function : MATLAB Function  TreatAsAtomicUnit=on
  Mux : Mux  Inputs=2
  wires:
  commands/1 -> MATLAB Function/6(cmds)
  Clock/1 -> MATLAB Function/1(time)
  altitude/1 -> MATLAB Function/2(h)
  VT/1 -> MATLAB Function/3(Vt)
  V3D/1 -> MATLAB Function/4(V3D)
  V3D_EKF/1 -> MATLAB Function/5(V3D_EKF)
  euler_XPlane/1 -> Mux/1
  euler_EKF/1 -> Mux/2
  Mux/1 -> MATLAB Function/7(euler)

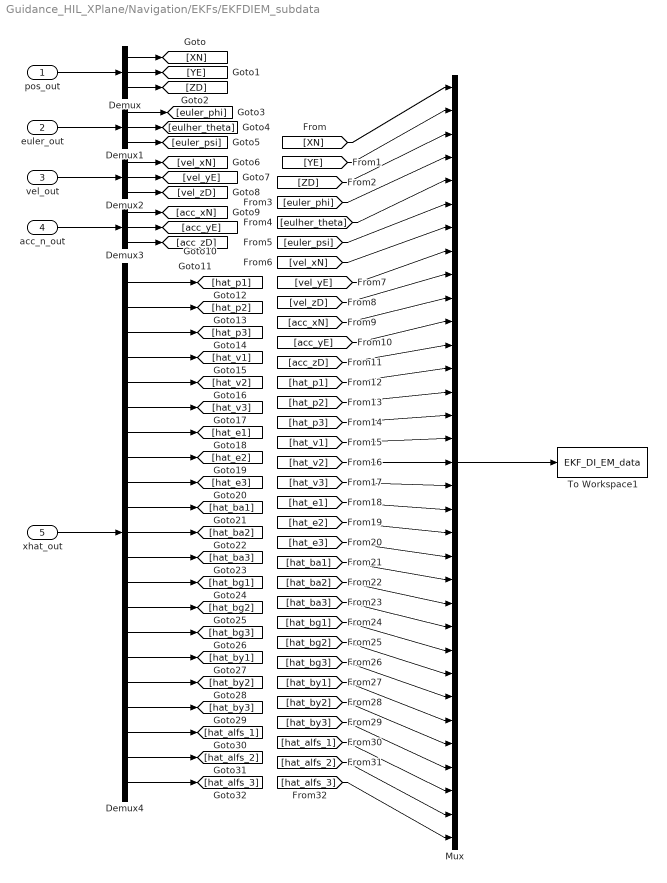
== system Guidance_HIL_XPlane/Navigation/EKFs/EKFDIEM_subdata ==
  pos_out : Inport
  euler_out : Inport  Port=2
  vel_out : Inport  Port=3
  acc_n_out : Inport  Port=4
  xhat_out : Inport  Port=5
  Demux{,1..3} (4 alike) : Demux  Outputs=3
  Demux4 : Demux  Outputs=21
  Mux : Mux  Inputs=33
  To Workspace1 : ToWorkspace  VariableName=EKF_DI_EM_data  SaveFormat=Structure With Time  SampleTime=-1
  wires:
  pos_out/1 -> Demux/1
  Demux/1 -> [XN]
  Demux/2 -> [YE]
  Demux/3 -> [ZD]
  Demux1/2 -> [eulher_theta]
  Demux1/1 -> [euler_phi]
  Demux1/3 -> [euler_psi]
  euler_out/1 -> Demux1/1
  Demux2/3 -> [vel_zD]
  Demux2/2 -> [vel_yE]
  Demux2/1 -> [vel_xN]
  vel_out/1 -> Demux2/1
  Demux3/3 -> [acc_zD]
  Demux3/1 -> [acc_xN]
  Demux3/2 -> [acc_yE]
  acc_n_out/1 -> Demux3/1
  xhat_out/1 -> Demux4/1
  Demux4/1 -> [hat_p1]
  Demux4/2 -> [hat_p2]
  Demux4/3 -> [hat_p3]
  Demux4/4 -> [hat_v1]
  Demux4/5 -> [hat_v2]
  Demux4/6 -> [hat_v3]
  Demux4/7 -> [hat_e1]
  Demux4/8 -> [hat_e2]
  Demux4/9 -> [hat_e3]
  Demux4/10 -> [hat_ba1]
  Demux4/11 -> [hat_ba2]
  Demux4/12 -> [hat_ba3]
  Demux4/13 -> [hat_bg1]
  Demux4/14 -> [hat_bg2]
  Demux4/15 -> [hat_bg3]
  Demux4/16 -> [hat_by1]
  Demux4/17 -> [hat_by2]
  Demux4/18 -> [hat_by3]
  Demux4/19 -> [hat_alfs_1]
  Demux4/20 -> [hat_alfs_2]
  Demux4/21 -> [hat_alfs_3]
  [XN] -> Mux/1
  [YE] -> Mux/2
  [ZD] -> Mux/3
  [euler_phi] -> Mux/4
  [eulher_theta] -> Mux/5
  [euler_psi] -> Mux/6
  [vel_xN] -> Mux/7
  [vel_yE] -> Mux/8
  [vel_zD] -> Mux/9
  [acc_xN] -> Mux/10
  [acc_yE] -> Mux/11
  [acc_zD] -> Mux/12
  [hat_p1] -> Mux/13
  [hat_p2] -> Mux/14
  [hat_p3] -> Mux/15
  [hat_v1] -> Mux/16
  [hat_v2] -> Mux/17
  [hat_v3] -> Mux/18
  [hat_e1] -> Mux/19
  [hat_e2] -> Mux/20
  [hat_e3] -> Mux/21
  [hat_ba1] -> Mux/22
  [hat_ba2] -> Mux/23
  [hat_ba3] -> Mux/24
  [hat_bg1] -> Mux/25
  [hat_bg2] -> Mux/26
  [hat_bg3] -> Mux/27
  [hat_by1] -> Mux/28
  [hat_by2] -> Mux/29
  [hat_by3] -> Mux/30
  [hat_alfs_1] -> Mux/31
  [hat_alfs_2] -> Mux/32
  [hat_alfs_3] -> Mux/33
  Mux/1 -> To Workspace1/1

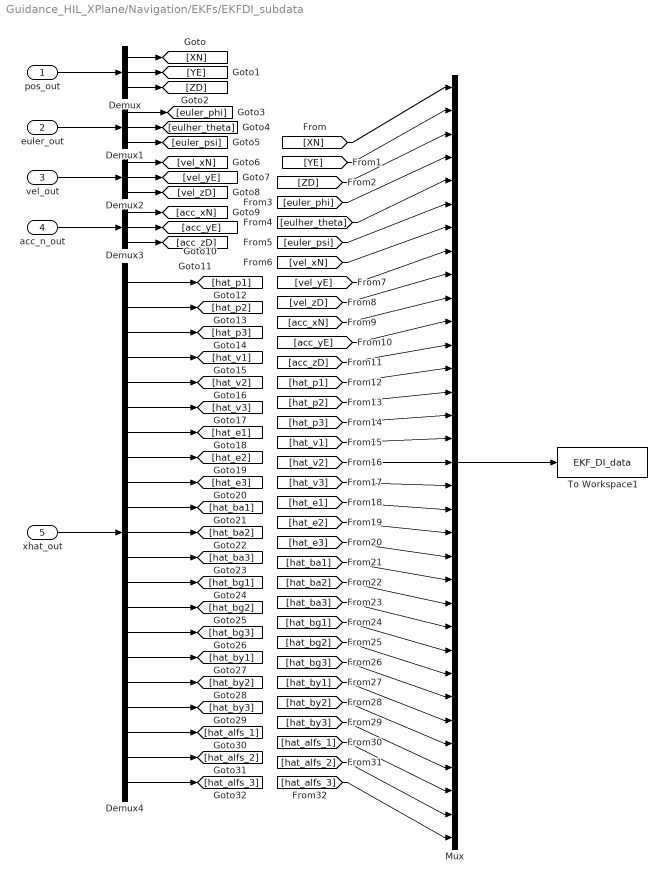
== system Guidance_HIL_XPlane/Navigation/EKFs/EKFDI_subdata ==
  pos_out : Inport
  euler_out : Inport  Port=2
  vel_out : Inport  Port=3
  acc_n_out : Inport  Port=4
  xhat_out : Inport  Port=5
  Demux{,1..3} (4 alike) : Demux  Outputs=3
  Demux4 : Demux  Outputs=21
  Mux : Mux  Inputs=33
  To Workspace1 : ToWorkspace  VariableName=EKF_DI_data  SaveFormat=Structure With Time  SampleTime=-1
  wires:
  pos_out/1 -> Demux/1
  Demux/1 -> [XN]
  Demux/2 -> [YE]
  Demux/3 -> [ZD]
  Demux1/2 -> [eulher_theta]
  Demux1/1 -> [euler_phi]
  Demux1/3 -> [euler_psi]
  euler_out/1 -> Demux1/1
  Demux2/3 -> [vel_zD]
  Demux2/2 -> [vel_yE]
  Demux2/1 -> [vel_xN]
  vel_out/1 -> Demux2/1
  Demux3/3 -> [acc_zD]
  Demux3/1 -> [acc_xN]
  Demux3/2 -> [acc_yE]
  acc_n_out/1 -> Demux3/1
  xhat_out/1 -> Demux4/1
  Demux4/1 -> [hat_p1]
  Demux4/2 -> [hat_p2]
  Demux4/3 -> [hat_p3]
  Demux4/4 -> [hat_v1]
  Demux4/5 -> [hat_v2]
  Demux4/6 -> [hat_v3]
  Demux4/7 -> [hat_e1]
  Demux4/8 -> [hat_e2]
  Demux4/9 -> [hat_e3]
  Demux4/10 -> [hat_ba1]
  Demux4/11 -> [hat_ba2]
  Demux4/12 -> [hat_ba3]
  Demux4/13 -> [hat_bg1]
  Demux4/14 -> [hat_bg2]
  Demux4/15 -> [hat_bg3]
  Demux4/16 -> [hat_by1]
  Demux4/17 -> [hat_by2]
  Demux4/18 -> [hat_by3]
  Demux4/19 -> [hat_alfs_1]
  Demux4/20 -> [hat_alfs_2]
  Demux4/21 -> [hat_alfs_3]
  [XN] -> Mux/1
  [YE] -> Mux/2
  [ZD] -> Mux/3
  [euler_phi] -> Mux/4
  [eulher_theta] -> Mux/5
  [euler_psi] -> Mux/6
  [vel_xN] -> Mux/7
  [vel_yE] -> Mux/8
  [vel_zD] -> Mux/9
  [acc_xN] -> Mux/10
  [acc_yE] -> Mux/11
  [acc_zD] -> Mux/12
  [hat_p1] -> Mux/13
  [hat_p2] -> Mux/14
  [hat_p3] -> Mux/15
  [hat_v1] -> Mux/16
  [hat_v2] -> Mux/17
  [hat_v3] -> Mux/18
  [hat_e1] -> Mux/19
  [hat_e2] -> Mux/20
  [hat_e3] -> Mux/21
  [hat_ba1] -> Mux/22
  [hat_ba2] -> Mux/23
  [hat_ba3] -> Mux/24
  [hat_bg1] -> Mux/25
  [hat_bg2] -> Mux/26
  [hat_bg3] -> Mux/27
  [hat_by1] -> Mux/28
  [hat_by2] -> Mux/29
  [hat_by3] -> Mux/30
  [hat_alfs_1] -> Mux/31
  [hat_alfs_2] -> Mux/32
  [hat_alfs_3] -> Mux/33
  Mux/1 -> To Workspace1/1

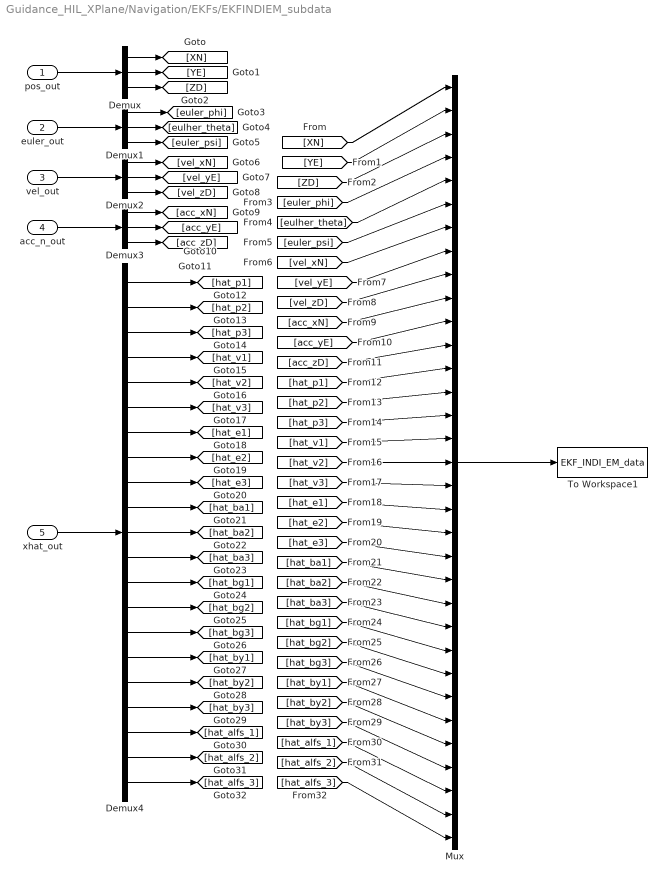
== system Guidance_HIL_XPlane/Navigation/EKFs/EKFINDIEM_subdata ==
  pos_out : Inport
  euler_out : Inport  Port=2
  vel_out : Inport  Port=3
  acc_n_out : Inport  Port=4
  xhat_out : Inport  Port=5
  Demux{,1..3} (4 alike) : Demux  Outputs=3
  Demux4 : Demux  Outputs=21
  Mux : Mux  Inputs=33
  To Workspace1 : ToWorkspace  VariableName=EKF_INDI_EM_data  SaveFormat=Structure With Time  SampleTime=-1
  wires:
  pos_out/1 -> Demux/1
  Demux/1 -> [XN]
  Demux/2 -> [YE]
  Demux/3 -> [ZD]
  Demux1/2 -> [eulher_theta]
  Demux1/1 -> [euler_phi]
  Demux1/3 -> [euler_psi]
  euler_out/1 -> Demux1/1
  Demux2/3 -> [vel_zD]
  Demux2/2 -> [vel_yE]
  Demux2/1 -> [vel_xN]
  vel_out/1 -> Demux2/1
  Demux3/3 -> [acc_zD]
  Demux3/1 -> [acc_xN]
  Demux3/2 -> [acc_yE]
  acc_n_out/1 -> Demux3/1
  xhat_out/1 -> Demux4/1
  Demux4/1 -> [hat_p1]
  Demux4/2 -> [hat_p2]
  Demux4/3 -> [hat_p3]
  Demux4/4 -> [hat_v1]
  Demux4/5 -> [hat_v2]
  Demux4/6 -> [hat_v3]
  Demux4/7 -> [hat_e1]
  Demux4/8 -> [hat_e2]
  Demux4/9 -> [hat_e3]
  Demux4/10 -> [hat_ba1]
  Demux4/11 -> [hat_ba2]
  Demux4/12 -> [hat_ba3]
  Demux4/13 -> [hat_bg1]
  Demux4/14 -> [hat_bg2]
  Demux4/15 -> [hat_bg3]
  Demux4/16 -> [hat_by1]
  Demux4/17 -> [hat_by2]
  Demux4/18 -> [hat_by3]
  Demux4/19 -> [hat_alfs_1]
  Demux4/20 -> [hat_alfs_2]
  Demux4/21 -> [hat_alfs_3]
  [XN] -> Mux/1
  [YE] -> Mux/2
  [ZD] -> Mux/3
  [euler_phi] -> Mux/4
  [eulher_theta] -> Mux/5
  [euler_psi] -> Mux/6
  [vel_xN] -> Mux/7
  [vel_yE] -> Mux/8
  [vel_zD] -> Mux/9
  [acc_xN] -> Mux/10
  [acc_yE] -> Mux/11
  [acc_zD] -> Mux/12
  [hat_p1] -> Mux/13
  [hat_p2] -> Mux/14
  [hat_p3] -> Mux/15
  [hat_v1] -> Mux/16
  [hat_v2] -> Mux/17
  [hat_v3] -> Mux/18
  [hat_e1] -> Mux/19
  [hat_e2] -> Mux/20
  [hat_e3] -> Mux/21
  [hat_ba1] -> Mux/22
  [hat_ba2] -> Mux/23
  [hat_ba3] -> Mux/24
  [hat_bg1] -> Mux/25
  [hat_bg2] -> Mux/26
  [hat_bg3] -> Mux/27
  [hat_by1] -> Mux/28
  [hat_by2] -> Mux/29
  [hat_by3] -> Mux/30
  [hat_alfs_1] -> Mux/31
  [hat_alfs_2] -> Mux/32
  [hat_alfs_3] -> Mux/33
  Mux/1 -> To Workspace1/1

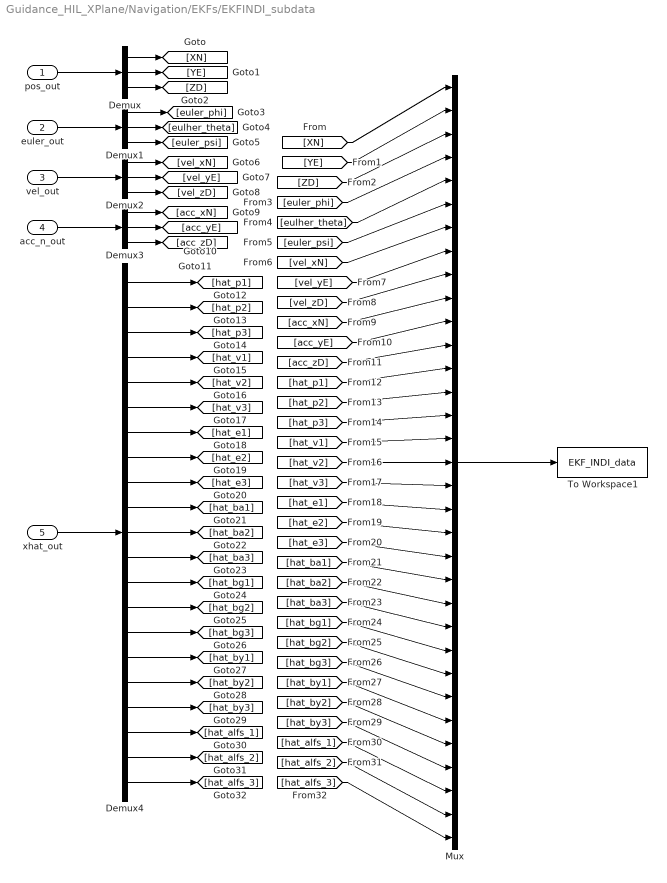
== system Guidance_HIL_XPlane/Navigation/EKFs/EKFINDI_subdata ==
  pos_out : Inport
  euler_out : Inport  Port=2
  vel_out : Inport  Port=3
  acc_n_out : Inport  Port=4
  xhat_out : Inport  Port=5
  Demux{,1..3} (4 alike) : Demux  Outputs=3
  Demux4 : Demux  Outputs=21
  Mux : Mux  Inputs=33
  To Workspace1 : ToWorkspace  VariableName=EKF_INDI_data  SaveFormat=Structure With Time  SampleTime=-1
  wires:
  pos_out/1 -> Demux/1
  Demux/1 -> [XN]
  Demux/2 -> [YE]
  Demux/3 -> [ZD]
  Demux1/2 -> [eulher_theta]
  Demux1/1 -> [euler_phi]
  Demux1/3 -> [euler_psi]
  euler_out/1 -> Demux1/1
  Demux2/3 -> [vel_zD]
  Demux2/2 -> [vel_yE]
  Demux2/1 -> [vel_xN]
  vel_out/1 -> Demux2/1
  Demux3/3 -> [acc_zD]
  Demux3/1 -> [acc_xN]
  Demux3/2 -> [acc_yE]
  acc_n_out/1 -> Demux3/1
  xhat_out/1 -> Demux4/1
  Demux4/1 -> [hat_p1]
  Demux4/2 -> [hat_p2]
  Demux4/3 -> [hat_p3]
  Demux4/4 -> [hat_v1]
  Demux4/5 -> [hat_v2]
  Demux4/6 -> [hat_v3]
  Demux4/7 -> [hat_e1]
  Demux4/8 -> [hat_e2]
  Demux4/9 -> [hat_e3]
  Demux4/10 -> [hat_ba1]
  Demux4/11 -> [hat_ba2]
  Demux4/12 -> [hat_ba3]
  Demux4/13 -> [hat_bg1]
  Demux4/14 -> [hat_bg2]
  Demux4/15 -> [hat_bg3]
  Demux4/16 -> [hat_by1]
  Demux4/17 -> [hat_by2]
  Demux4/18 -> [hat_by3]
  Demux4/19 -> [hat_alfs_1]
  Demux4/20 -> [hat_alfs_2]
  Demux4/21 -> [hat_alfs_3]
  [XN] -> Mux/1
  [YE] -> Mux/2
  [ZD] -> Mux/3
  [euler_phi] -> Mux/4
  [eulher_theta] -> Mux/5
  [euler_psi] -> Mux/6
  [vel_xN] -> Mux/7
  [vel_yE] -> Mux/8
  [vel_zD] -> Mux/9
  [acc_xN] -> Mux/10
  [acc_yE] -> Mux/11
  [acc_zD] -> Mux/12
  [hat_p1] -> Mux/13
  [hat_p2] -> Mux/14
  [hat_p3] -> Mux/15
  [hat_v1] -> Mux/16
  [hat_v2] -> Mux/17
  [hat_v3] -> Mux/18
  [hat_e1] -> Mux/19
  [hat_e2] -> Mux/20
  [hat_e3] -> Mux/21
  [hat_ba1] -> Mux/22
  [hat_ba2] -> Mux/23
  [hat_ba3] -> Mux/24
  [hat_bg1] -> Mux/25
  [hat_bg2] -> Mux/26
  [hat_bg3] -> Mux/27
  [hat_by1] -> Mux/28
  [hat_by2] -> Mux/29
  [hat_by3] -> Mux/30
  [hat_alfs_1] -> Mux/31
  [hat_alfs_2] -> Mux/32
  [hat_alfs_3] -> Mux/33
  Mux/1 -> To Workspace1/1

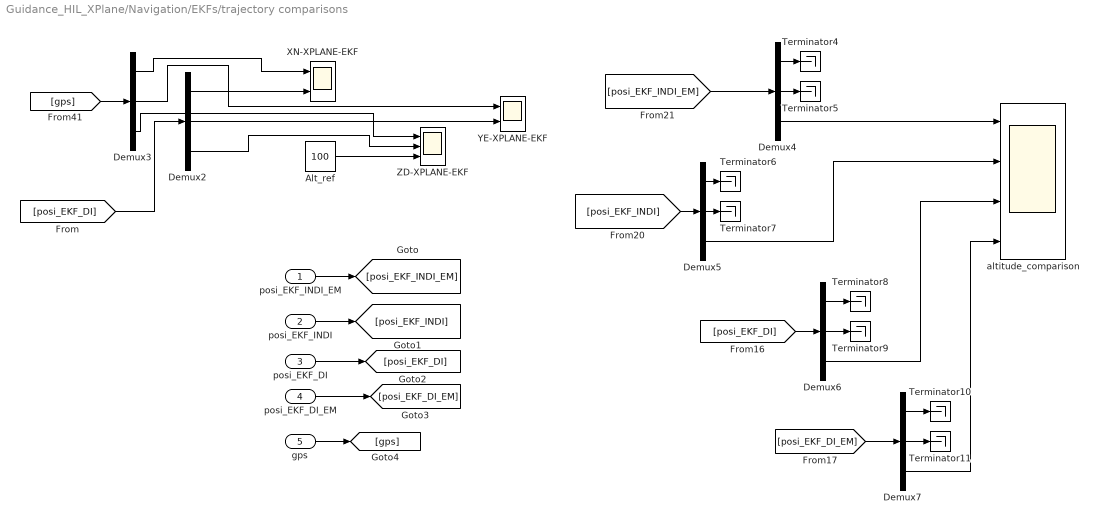
== system Guidance_HIL_XPlane/Navigation/EKFs/trajectory comparisons ==
  posi_EKF_INDI_EM : Inport
  posi_EKF_INDI : Inport  Port=2
  posi_EKF_DI : Inport  Port=3
  posi_EKF_DI_EM : Inport  Port=4
  gps : Inport  Port=5
  Alt_ref : Constant  Value=100
  Demux{2..7} (6 alike) : Demux  Outputs=3
  Terminator{4..11} (8 alike) : Terminator
  XN-XPLANE-EKF : Scope  NumInputPorts=2
      settings: ActiveDisplayYMinimum=-162.600711820487  ActiveDisplayYMaximum=541.8471053905007  DataLoggingVariableName=ScopeData14
  YE-XPLANE-EKF : Scope  NumInputPorts=2
      settings: ActiveDisplayYMinimum=-323.45260691868168  ActiveDisplayYMaximum=717.33765548501469  DataLoggingVariableName=ScopeData12
  ZD-XPLANE-EKF : Scope  NumInputPorts=3
      settings: ActiveDisplayYMinimum=-291.51496653616971  ActiveDisplayYMaximum=162.5783774481977  DataLoggingVariableName=ScopeData15
  altitude_comparison : Scope  NumInputPorts=4
      settings: ActiveDisplayYMinimum=-177.02475407024423  ActiveDisplayYMaximum=323.613157672522  DataLoggingVariableName=ScopeData19
  wires:
  posi_EKF_INDI_EM/1 -> [posi_EKF_INDI_EM]
  Demux6/1 -> Terminator8/1
  Demux5/3 -> altitude_comparison/2
  Demux5/2 -> Terminator7/1
  [posi_EKF_INDI_EM] -> Demux4/1
  Demux7/1 -> Terminator10/1
  Demux5/1 -> Terminator6/1
  [posi_EKF_DI] -> Demux6/1
  Demux6/3 -> altitude_comparison/3
  Demux4/2 -> Terminator5/1
  Demux7/3 -> altitude_comparison/4
  Demux4/3 -> altitude_comparison/1
  [posi_EKF_DI_EM] -> Demux7/1
  Demux6/2 -> Terminator9/1
  Demux4/1 -> Terminator4/1
  Demux7/2 -> Terminator11/1
  [posi_EKF_INDI] -> Demux5/1
  posi_EKF_INDI/1 -> [posi_EKF_INDI]
  posi_EKF_DI/1 -> [posi_EKF_DI]
  posi_EKF_DI_EM/1 -> [posi_EKF_DI_EM]
  Demux3/3 -> ZD-XPLANE-EKF/1
  Demux3/2 -> YE-XPLANE-EKF/1
  Demux2/3 -> ZD-XPLANE-EKF/2
  [posi_EKF_DI] -> Demux2/1
  [gps] -> Demux3/1
  Demux3/1 -> XN-XPLANE-EKF/1
  Alt_ref/1 -> ZD-XPLANE-EKF/3
  Demux2/1 -> XN-XPLANE-EKF/2
  Demux2/2 -> YE-XPLANE-EKF/2
  gps/1 -> [gps]

== system Guidance_HIL_XPlane/Navigation/Error_Modeling/GPSNEO8M1 ==
  pos_ned_true : Inport
  vel_ned_true : Inport  Port=2
  time : Inport  Port=3
  GPSNoise_bias : Subsystem
  GPSNoise_pos : Subsystem
  GPSNoise_vel : Subsystem
  MATLAB Function : MATLAB Function  TreatAsAtomicUnit=on
  pos_em : Outport
  vel_em : Outport  Port=2
  wires:
  MATLAB Function/1(pos_em) -> pos_em/1
  MATLAB Function/2(vel_em) -> vel_em/1
  pos_ned_true/1 -> MATLAB Function/1(pos_ned_true)
  vel_ned_true/1 -> MATLAB Function/2(vel_ned_true)
  time/1 -> MATLAB Function/3(t)
  GPSNoise_pos/1(noise_pos) -> MATLAB Function/4(noise_pos_m)
  GPSNoise_vel/1(noise_vel) -> MATLAB Function/5(noise_vel_ms)
  GPSNoise_bias/1(noise_bias) -> MATLAB Function/6(w_bias_pos)

== system Guidance_HIL_XPlane/Navigation/Error_Modeling/ICM20689 ==
  pqr : Inport
  acc : Inport  Port=2
  Temperature : Inport  Port=3
  AccNoise_ms2 : Subsystem
  Gain : Gain  Gain=180/pi
  Gain1 : Gain  Gain=pi/180
  Gain2 : Gain  Gain=180/pi
  Gain3 : Gain  Gain=pi/180
  GyroNoise_dps : Subsystem
  Reshape : Reshape  OutputDimensionality=Customize  OutputDimensions=[3 1]
  Reshape1 : Reshape  OutputDimensionality=Customize  OutputDimensions=[3 1]
  acc_core : MATLAB Function  TreatAsAtomicUnit=on
  gyro_core : MATLAB Function  TreatAsAtomicUnit=on
  pqr_meas_ins : Outport
  acc_meas_ins : Outport  Port=2
  wires:
  pqr/1 -> Gain/1
  Gain/1 -> gyro_core/1(omega_true_dps)
  Temperature/1 -> acc_core/2(T), gyro_core/2(T)
  acc/1 -> Gain2/1
  Gain2/1 -> acc_core/1(acc_true_ms2)
  acc_core/1(acc_meas_ms2) -> Gain3/1
  Gain3/1 -> acc_meas_ins/1
  GyroNoise_dps/1(noise_dps) -> Reshape/1
  Reshape/1 -> gyro_core/3(noise_dps)
  AccNoise_ms2/1(noise_dps) -> Reshape1/1
  Reshape1/1 -> acc_core/3(noise_ms2)
  gyro_core/1(omega_meas_dps) -> pqr_meas_ins/1

== system Guidance_HIL_XPlane/Navigation/Error_Modeling/MAG-IST8310 ==
  euler_in : Inport
  temperature : Inport  Port=2
  mag_var_xplane : Inport  Port=3
  Demux : Demux  Outputs=3
  IST8320-Noise : Subsystem
  MATLAB Function : MATLAB Function  TreatAsAtomicUnit=on
  Mux1 : Mux  Inputs=3
  Terminator : Terminator
  eul_em : Outport
  wires:
  euler_in/1 -> MATLAB Function/1(euler_true_rad), Demux/1
  Mux1/1 -> eul_em/1
  Demux/1 -> Mux1/1
  Demux/2 -> Mux1/2
  MATLAB Function/1(yaw_mag_rad) -> Mux1/3
  temperature/1 -> MATLAB Function/2(T)
  IST8320-Noise/1(noise_yaw) -> MATLAB Function/3(noise_mag_uT)
  Demux/3 -> Terminator/1
  mag_var_xplane/1 -> MATLAB Function/4(mag_var)

== system Guidance_HIL_XPlane/Navigation/Error_Modeling/GPSNEO8M1/GPSNoise_bias ==
  Mux : Mux  Inputs=3
  Random Number : RandomNumber  Seed=sensors.gps.noise_seed_bias(1)  SampleTime=sensors.gps.Ts
  Random Number1 : RandomNumber  Seed=sensors.gps.noise_seed_bias(3)  SampleTime=sensors.gps.Ts
  Random Number2 : RandomNumber  Seed=sensors.gps.noise_seed_bias(2)  SampleTime=sensors.gps.Ts
  noise_bias : Outport
  wires:
  Random Number/1 -> Mux/1
  Random Number2/1 -> Mux/2
  Random Number1/1 -> Mux/3
  Mux/1 -> noise_bias/1

== system Guidance_HIL_XPlane/Navigation/Error_Modeling/GPSNEO8M1/GPSNoise_pos ==
  Mux : Mux  Inputs=3
  Random Number : RandomNumber  Variance=sensors.gps.sigma_eta_pos_NED(1)^2  Seed=sensors.gps.noise_seed_pos(1)  SampleTime=sensors.gps.Ts
  Random Number1 : RandomNumber  Variance=sensors.gps.sigma_eta_pos_NED(3)^2  Seed=sensors.gps.noise_seed_pos(3)  SampleTime=sensors.gps.Ts
  Random Number2 : RandomNumber  Variance=sensors.gps.sigma_eta_pos_NED(2)^2  Seed=sensors.gps.noise_seed_pos(2)  SampleTime=sensors.gps.Ts
  noise_pos : Outport
  wires:
  Random Number/1 -> Mux/1
  Random Number2/1 -> Mux/2
  Random Number1/1 -> Mux/3
  Mux/1 -> noise_pos/1

== system Guidance_HIL_XPlane/Navigation/Error_Modeling/GPSNEO8M1/GPSNoise_vel ==
  Mux : Mux  Inputs=3
  Random Number : RandomNumber  Variance=sensors.gps.sigma_vel_NED(1)^2  Seed=sensors.gps.noise_seed_vel(1)  SampleTime=sensors.gps.Ts
  Random Number1 : RandomNumber  Variance=sensors.gps.sigma_vel_NED(3)^2  Seed=sensors.gps.noise_seed_vel(3)  SampleTime=sensors.gps.Ts
  Random Number2 : RandomNumber  Variance=sensors.gps.sigma_vel_NED(2)^2  Seed=sensors.gps.noise_seed_vel(2)  SampleTime=sensors.gps.Ts
  noise_vel : Outport
  wires:
  Random Number/1 -> Mux/1
  Random Number2/1 -> Mux/2
  Random Number1/1 -> Mux/3
  Mux/1 -> noise_vel/1

== system Guidance_HIL_XPlane/Navigation/Error_Modeling/ICM20689/AccNoise_ms2 ==
  Mux : Mux  Inputs=3
  Random Number : RandomNumber  Variance=sensors.icm20689.acc.sigma_noise_ms2^2  Seed=sensors.seeds.icm20689.acc.noise(1)  SampleTime=sensors.sys.Ts
  Random Number1 : RandomNumber  Variance=sensors.icm20689.acc.sigma_noise_ms2^2  Seed=sensors.seeds.icm20689.acc.noise(3)  SampleTime=sensors.sys.Ts
  Random Number2 : RandomNumber  Variance=sensors.icm20689.acc.sigma_noise_ms2^2  Seed=sensors.seeds.icm20689.acc.noise(2)  SampleTime=sensors.sys.Ts
  noise_dps : Outport
  wires:
  Random Number/1 -> Mux/1
  Random Number2/1 -> Mux/2
  Random Number1/1 -> Mux/3
  Mux/1 -> noise_dps/1

== system Guidance_HIL_XPlane/Navigation/Error_Modeling/ICM20689/GyroNoise_dps ==
  Mux : Mux  Inputs=3
  Random Number : RandomNumber  Variance=sensors.icm20689.gyro.sigma_noise_dps^2  Seed=sensors.seeds.icm20689.gyro.noise(1)  SampleTime=sensors.sys.Ts
  Random Number1 : RandomNumber  Variance=sensors.icm20689.gyro.sigma_noise_dps^2  Seed=sensors.seeds.icm20689.gyro.noise(3)  SampleTime=sensors.sys.Ts
  Random Number2 : RandomNumber  Variance=sensors.icm20689.gyro.sigma_noise_dps^2  Seed=sensors.seeds.icm20689.gyro.noise(2)  SampleTime=sensors.sys.Ts
  noise_dps : Outport
  wires:
  Random Number/1 -> Mux/1
  Random Number2/1 -> Mux/2
  Random Number1/1 -> Mux/3
  Mux/1 -> noise_dps/1

== system Guidance_HIL_XPlane/Navigation/Error_Modeling/MAG-IST8310/IST8320-Noise ==
  Mux : Mux  Inputs=3
  Random Number : RandomNumber  Variance=sensors.ist8310.mag.sigma_noise_uT^2  Seed=sensors.seeds.ist8310.mag.noise(1)  SampleTime=sensors.ist8310.mag.Ts
  Random Number1 : RandomNumber  Variance=sensors.ist8310.mag.sigma_noise_uT^2  Seed=sensors.seeds.ist8310.mag.noise(3)  SampleTime=sensors.ist8310.mag.Ts
  Random Number2 : RandomNumber  Variance=sensors.ist8310.mag.sigma_noise_uT^2  Seed=sensors.seeds.ist8310.mag.noise(2)  SampleTime=sensors.ist8310.mag.Ts
  noise_yaw : Outport
  wires:
  Random Number/1 -> Mux/1
  Random Number2/1 -> Mux/2
  Random Number1/1 -> Mux/3
  Mux/1 -> noise_yaw/1

== matlab function Guidance_HIL_XPlane/Navigation/EKFs/MATLAB Function ==
  data: vN input; VT output; vE input; vD input
function VT  = true_air_speed(vN, vE, vD)
    VT = sqrt(vN^2 + vE^2 + vD^2);
end

== matlab function Guidance_HIL_XPlane/Navigation/EKFs/EKF_DIRETO_EM ==
  data: acc_b_in input; euler_out output; vel_out output; pos_out output; gyro_b_in input; pos_meas_in input; vel_meas_in input; eul_meas_in input; reset input; sample_valid input; t_now input; acc_n_out output; xhat_out output
function [euler_out, vel_out, pos_out, acc_n_out, xhat_out] = EKF_DI_EM_block( ...
    acc_b_in, gyro_b_in, pos_meas_in, vel_meas_in, eul_meas_in, reset, sample_valid, t_now)
%#codegen

coder.extrinsic('EKF_DI_EM_solver');
coder.extrinsic('evalin');

%% Saídas com dimensão fixa

euler_out = zeros(3,1);
vel_out   = zeros(3,1);
pos_out   = zeros(3,1);
acc_n_out = zeros(3,1);
xhat_out  = zeros(21,1);

%% Temporários com dimensão fixa

euler_tmp = zeros(3,1);
vel_tmp   = zeros(3,1);
pos_tmp   = zeros(3,1);
acc_tmp   = zeros(3,1);
xhat_tmp  = zeros(21,1);

%% Carrega parâmetros do workspace

EKF_DI_params = evalin('base', 'EKF_DI_params');

%% Chama solver externo

[euler_tmp, vel_tmp, pos_tmp, acc_tmp, xhat_tmp] = EKF_DI_EM_solver( ...
    acc_b_in, gyro_b_in, pos_meas_in, vel_meas_in, eul_meas_in, ...
    reset, sample_valid, t_now, EKF_DI_params);

%% Cópia elemento a elemento para forçar dimensão no Simulink

euler_out(1) = euler_tmp(1);
euler_out(2) = euler_tmp(2);
euler_out(3) = euler_tmp(3);

vel_out(1) = vel_tmp(1);
vel_out(2) = vel_tmp(2);
vel_out(3) = vel_tmp(3);

pos_out(1) = pos_tmp(1);
pos_out(2) = pos_tmp(2);
pos_out(3) = pos_tmp(3);

acc_n_out(1) = acc_tmp(1);
acc_n_out(2) = acc_tmp(2);
acc_n_out(3) = acc_tmp(3);

for k = 1:21
    xhat_out(k) = xhat_tmp(k);
end

end

== matlab function Guidance_HIL_XPlane/Navigation/EKFs/EKF_INDIRETO ==
  data: acc_b_in input; euler_out output; vel_out output; pos_out output; gyro_b_in input; pos_meas_in input; vel_meas_in input; eul_meas_in input; reset input; sample_valid input; t_now input; acc_n_out output; xhat_out output
function [euler_out, vel_out, pos_out, acc_n_out, xhat_out] = EKF_INDI_block( ...
    acc_b_in, gyro_b_in, pos_meas_in, vel_meas_in, eul_meas_in, reset, sample_valid, t_now)
%#codegen

coder.extrinsic('EKF_INDI_solver');
coder.extrinsic('evalin');

%% Saídas com dimensão fixa

euler_out = zeros(3,1);
vel_out   = zeros(3,1);
pos_out   = zeros(3,1);
acc_n_out = zeros(3,1);
xhat_out  = zeros(21,1);

%% Variáveis temporárias com dimensão fixa

euler_tmp = zeros(3,1);
vel_tmp   = zeros(3,1);
pos_tmp   = zeros(3,1);
acc_tmp   = zeros(3,1);
xhat_tmp  = zeros(21,1);

%% Carrega parâmetros do workspace

EKF_INDI_params = evalin('base', 'EKF_INDI_params');

%% Chama solver externo

[euler_tmp, vel_tmp, pos_tmp, acc_tmp, xhat_tmp] = EKF_INDI_solver( ...
    acc_b_in, gyro_b_in, pos_meas_in, vel_meas_in, eul_meas_in, ...
    reset, sample_valid, t_now, EKF_INDI_params);

%% Cópia elemento a elemento para forçar dimensão no Simulink

euler_out(1) = euler_tmp(1);
euler_out(2) = euler_tmp(2);
euler_out(3) = euler_tmp(3);

vel_out(1) = vel_tmp(1);
vel_out(2) = vel_tmp(2);
vel_out(3) = vel_tmp(3);

pos_out(1) = pos_tmp(1);
pos_out(2) = pos_tmp(2);
pos_out(3) = pos_tmp(3);

acc_n_out(1) = acc_tmp(1);
acc_n_out(2) = acc_tmp(2);
acc_n_out(3) = acc_tmp(3);

for k = 1:21
    xhat_out(k) = xhat_tmp(k);
end

end

== matlab function Guidance_HIL_XPlane/Navigation/EKFs/EKF_INDIRETO_EM ==
  data: acc_b_in input; euler_out output; vel_out output; pos_out output; gyro_b_in input; pos_meas_in input; vel_meas_in input; eul_meas_in input; reset input; sample_valid input; t_now input; acc_n_out output; xhat_out output
function [euler_out, vel_out, pos_out, acc_n_out, xhat_out] = EKF_INDI_EM_block( ...
    acc_b_in, gyro_b_in, pos_meas_in, vel_meas_in, eul_meas_in, reset, sample_valid, t_now)
%#codegen

coder.extrinsic('EKF_INDI_EM_solver');
coder.extrinsic('evalin');

%% Saídas com dimensão fixa

euler_out = zeros(3,1);
vel_out   = zeros(3,1);
pos_out   = zeros(3,1);
acc_n_out = zeros(3,1);
xhat_out  = zeros(21,1);

%% Variáveis temporárias com dimensão fixa

euler_tmp = zeros(3,1);
vel_tmp   = zeros(3,1);
pos_tmp   = zeros(3,1);
acc_tmp   = zeros(3,1);
xhat_tmp  = zeros(21,1);

%% Carrega parâmetros do workspace

EKF_INDI_params = evalin('base', 'EKF_INDI_params');

%% Chama solver externo

[euler_tmp, vel_tmp, pos_tmp, acc_tmp, xhat_tmp] = EKF_INDI_EM_solver( ...
    acc_b_in, gyro_b_in, pos_meas_in, vel_meas_in, eul_meas_in, ...
    reset, sample_valid, t_now, EKF_INDI_params);

%% Cópia elemento a elemento para forçar dimensão no Simulink

euler_out(1) = euler_tmp(1);
euler_out(2) = euler_tmp(2);
euler_out(3) = euler_tmp(3);

vel_out(1) = vel_tmp(1);
vel_out(2) = vel_tmp(2);
vel_out(3) = vel_tmp(3);

pos_out(1) = pos_tmp(1);
pos_out(2) = pos_tmp(2);
pos_out(3) = pos_tmp(3);

acc_n_out(1) = acc_tmp(1);
acc_n_out(2) = acc_tmp(2);
acc_n_out(3) = acc_tmp(3);

for k = 1:21
    xhat_out(k) = xhat_tmp(k);
end

end
